simulink model "drone_controller_config"  (R2026b)
settings: Solver=FixedStepDiscrete  StopTime=1  FixedStep=0.002
PreLoadFcn:
  | if ~bdIsLoaded('drone_controller')
  |     load_system(fullfile(fileparts(get_param(bdroot,'FileName')), 'drone_controller.slx'));
  | end
settings Model: Creator=ASUS  LastModifiedBy=ASUS

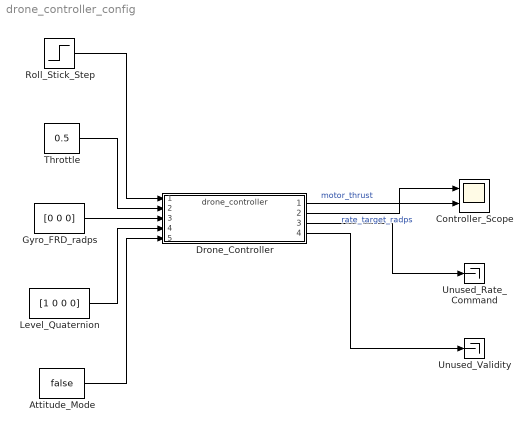
== system drone_controller_config ==
  Attitude_Mode : Constant  Value=false
  Controller_Scope : Scope  NumInputPorts=2
      settings: TimeSpan=1  Title=Body rate target (roll, pitch, yaw)  ActiveDisplayYMinimum=-0.56122429186550793  ActiveDisplayYMaximum=1.8146936274617713  YLabel=rad/s  DataLoggingVariableName=controller_demo_signals
  Drone_Controller : ModelReference  ModelNameDialog=drone_controller  SimulationMode=Normal  ModelReferenceVersion=1.6
  Gyro_FRD_radps : Constant  Value=[0 0 0]
  Level_Quaternion : Constant  Value=[1 0 0 0]
  Roll_Stick_Step : Step  Time=0.2  InitialValue=[0 0 0]  FinalValue=[0.5 0 0]  SampleTime=0.002
  Throttle : Constant  Value=0.5
  Unused_Rate_Command : Terminator
  Unused_Validity : Terminator
  wires:
  Drone_Controller/4 -> Unused_Validity/1
  Drone_Controller/3 -> Unused_Rate_Command/1
  Drone_Controller/2 -> Controller_Scope/1  "rate_target_radps"
  Drone_Controller/1 -> Controller_Scope/2  "motor_thrust"
  Attitude_Mode/1 -> Drone_Controller/5
  Level_Quaternion/1 -> Drone_Controller/4
  Gyro_FRD_radps/1 -> Drone_Controller/3
  Throttle/1 -> Drone_Controller/2
  Roll_Stick_Step/1 -> Drone_Controller/1
